simulink model "TP9_commande_ceintures_airbags"  (R2022b)
settings: Solver=VariableStepAuto  StartTime=0.0  StopTime=inf  RelTol=1e-3
libraries: dspsnks4 x2
settings Model: Creator=HP  LastModifiedBy=HP

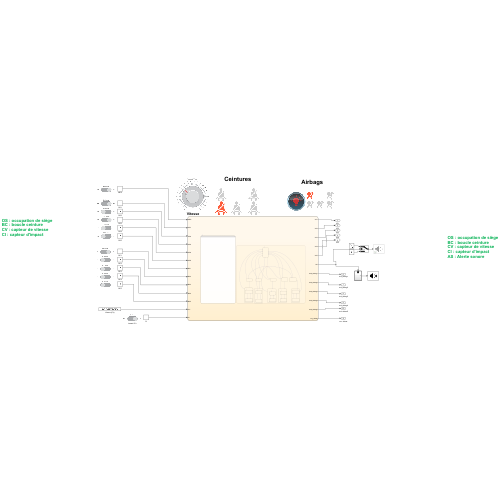
[thumbnail: Simulink's stored preview of the top-level diagram]
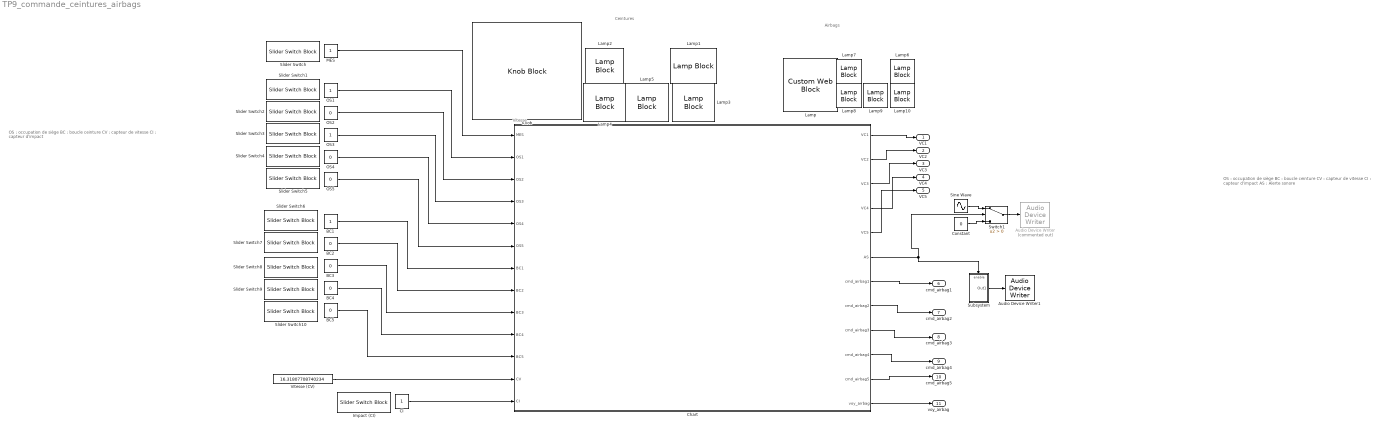
== system TP9_commande_ceintures_airbags ==
  note: Ceintures
  note: OS : occupation de siège
      | BC : boucle ceinture
      | CV : capteur de vitesse
      | CI : capteur d'impact
  note: OS : occupation de siège
      | BC : boucle ceinture
      | CV : capteur de vitesse
      | CI : capteur d'impact
      | AS : Alerte sonore
  note: Airbags
  note: Vitesse
  Audio Device Writer : dspsnks4/Audio Device Writer  Commented=on  Driver=DirectSound  Device=Default  InheritSampleRate=on  SampleRate=44100  BitDepth=16-bit integer  BufferSize=4096  NumBuffers=10  DefaultOutputChannelMapping=on  OutputChannelMapping=1:2  OutputNumUnderrunSamples=off  DriverIdx=1  DeviceWarnFlag=''
  Audio Device Writer1 : dspsnks4/Audio Device Writer  Driver=DirectSound  Device=Default  InheritSampleRate=on  SampleRate=44100  BitDepth=16-bit integer  BufferSize=4096  NumBuffers=10  DefaultOutputChannelMapping=on  OutputChannelMapping=1:2  OutputNumUnderrunSamples=off  DriverIdx=1  DeviceWarnFlag=''
  BC1 : Constant
  BC{2..5} (4 alike) : Constant  Value=0
  CI : Constant
  Chart : Stateflow chart  TreatAsAtomicUnit=on
      settings: PortSchema="{\"entries\":[{\"content\":{\"sides\":[{\"content\":{\"connectorIds\":[\"In1\",\"In2\",\"In3\",\"In4\",\"In5\",\"In6\",\"In7\",\"In8\",\"In9\",\"In10\",\"In12\",\"In11\",\"In13\"]},\"type\":\"ConnectorPlacement.EquallySpacedRectSide\",\"uuid\":\"46ff6330-a002-4d17-9cd2-f1bd6e651efc\"},{\"content\":{\"connectorIds\":[\"Out1\",\"Out2\",\"Out3\",\"Out4\",\"Out5\",\"Out6\",\"Out7\",\"Out8\",\"Out9\",\"Out10\",\"Out11\",\"Out12\"],\"side\":\"RIGHT\"},\"type\":\"ConnectorPlacement.EquallySpacedRectSide\",\"uuid\":\"880f7646-c9e2-4dea-b189-cc9f9386497e\"},{\"content\":{\"connectorIds\":[],\"side\":\"TOP\"},\"type\":\"ConnectorPlacement.EquallySpacedRectSide\",\"uuid\":\"9bbd1801-2f42-4ba2-a8a0-b1f6ca3d8990\"}]},\"type\":\"ConnectorPlacement.EquallySpacedConnector\",\"uuid\":\"8416df3d-9e50-44e6-a163-5e155c7c1857\"}],\"packageUris\":[\"http://schema.mathworks.com/mf0/Connector/R2020b\"],\"version\":\"1.0\"}"
  Constant : Constant  Value=0
  Impact (CI) : SliderSwitchBlock
      settings: Values={{'Off', 'On'}, [0 1]}
  Knob : KnobBlock  ScaleMax=50
  Lamp : CustomWebBlock  LabelPosition=Hide  ShowInitialText=on  Configuration="{\"components\":[{\"name\":\"BackgroundImageComponent\",\"settings\":{\"image\":{\"size\":[150,150],\"src\":\"data:image\\/svg+xml;base64,PHN2ZyB4bWxucz0iaHR0cDovL3d3dy53My5vcmcvMjAwMC9zdmciIHhtbG5zOnhsaW5rPSJodHRwOi8vd3d3LnczLm9yZy8xOTk5L3hsaW5rIiB2aWV3Qm94PSIwIDAgNTAwIDUwMCI+PGRlZnM+PHN0eWxlPi5he2ZpbGw6dXJsKCNhKTt9LmJ7ZmlsbDp1cmwoI2IpO30uY3tmaWxsOnVybCgjYyk7fTwvc3R5bGU+PHJhZGlhbEdyYWRpZW50IGlkPSJhIiBjeD0iMjgzLjg0IiBjeT0iLTQ2Ni4zNyIgcj0iMzc1Ljc1IiBncmFkaWVudFRyYW5zZm9ybT0ibWF0cml4KDEuMzksIDAsIDAsIC0xLjM5LCAtMTUzLjU2LCAtNjQ0LjA4KSIg ...(+2088 chars)\",\"srcOrientation\":\"Right\"},\"position\":[0,0,1,1],\"scaleMode\":\"0\"}},{\"name\":\"LampStateComponent\",\"settings\":{\"position\":[0,0,1,1],\"states\":[{\"icon\":{\"customSrc\":\"data:image\\/svg+xml;base64,PHN2ZyBpZD0iTGF5ZXJfMSIgZGF0YS1uYW1lPSJMYXllciAxIiB4bWxucz0iaHR0cDovL3d3dy53My5vcmcvMjAwMC9zdmciIHZpZXdCb3g9IjAgMCA0MTEgNDU4Ij48ZGVmcz48c3R5bGU+LmNscy0xe2ZpbGw6I2ZkZjhjMTt9LmNscy0ye2ZpbGw6I2ZlZTEwMDt9LmNscy0ze2ZpbGw6IzIzMWYyMDt9LmNscy00e2ZpbGw6I2EwOWY5Zjt9LmNscy00LC5jbHMtNSwuY2xzLTZ7c3Ryb2tlOiMyMzFmMjA7c3Ryb2tlLW1pdGVybGltaXQ6MTA7fS5jbHMtNXtmaWxsOiNmZmY7fS5jbHMtNntmaWxsOm5vbmU7fTwvc3R5bGU+PC9kZWZz ...(+5168 chars)\",\"id\":-1,\"srcOrientation\":\"Right\",\"type\":\"custom\"},\"iconScale\":0.8,\"metadata\":{},\"overlayType\":\"intersect\",\"shape\":{\"color\":[0.725,0,0],\"opacity\":1,\"position\":[0.1,0.1,0.8,0.8],\"type\":\"ellipse\"},\"value\":[]},{\"icon\":{\"customSrc\":\"data:image\\/svg+xml;base64,PHN2ZyBpZD0iTGF5ZXJfMSIgZGF0YS1uYW1lPSJMYXllciAxIiB4bWxucz0iaHR0cDovL3d3dy53My5vcmcvMjAwMC9zdmciIHZpZXdCb3g9IjAgMCA0MTEgNDU4Ij48ZGVmcz48c3R5bGU+LmNscy0xe2ZpbGw6I2ZkZjhjMTt9LmNscy0ye2ZpbGw6I2ZlZTEwMDt9LmNscy0ze2ZpbGw6IzIzMWYyMDt9LmNscy00e2ZpbGw6I2EwOWY5Zjt9LmNscy00LC5jbHMtNSwuY2xzLTZ7c3Ryb2tlOiMyMzFmMjA7c3Ryb2tlLW1pdGVybGltaXQ6MTA7fS5jbHMtNXtmaWxsOiNmZmY7fS5jbHMtNntmaWxsOm5vbmU7fTwvc3R5bGU+PC9kZWZz ...(+5168 chars)\",\"id\":-1,\"srcOrientation\":\"Right\",\"type\":\"custom\"},\"iconScale\":0.8,\"metadata\":{\"useDefaults\":{\"customIcon\":true,\"icon\":true,\"overlayType\":true,\"shape\":true,\"sizeAndPosition\":true}},\"overlayType\":\"intersect\",\"shape\":{\"color\":[0,0,0],\"opacity\":1,\"position\":[0.1,0.1,0.8,0.8],\"type\":\"ellipse\"},\"value\":\"0\"}],\"valueType\":\"discrete\"}},{\"name\":\"ForegroundImageComponent\",\"settings\":{\"image\":{\"size\":[150,150],\"src\":\"data:image\\/svg+xml;base64,PHN2ZyB4bWxucz0iaHR0cDovL3d3dy53My5vcmcvMjAwMC9zdmciIHhtbG5zOnhsaW5rPSJodHRwOi8vd3d3LnczLm9yZy8xOTk5L3hsaW5rIiB2aWV3Qm94PSIwIDAgNTAwIDUwMCI+PGRlZnM+PHN0eWxlPi5he2ZpbGw6dXJsKCNhKTt9PC9zdHlsZT48bGluZWFyR3JhZGllbnQgaWQ9ImEiIHgxPSIxNzMuMDUiIHkxPSItNjI3Ljc4IiB4Mj0iMTczLjA1IiB5Mj0iLTUyMi40MyIgZ3JhZGllbnRUcmFuc2Zvcm09Im1hdHJpeCgxLjI5LCAwLCAwLCAtMS4zMywgMjcuMTMsIC02MjguMzEpIiBncmFkaWVudFVuaXRzPSJ1c2VyU3BhY2VPblVzZSI+PHN0b3Agb2Zmc2V0PSIwIiBzdG9wLWNvbG9yPSIjZmZmIiBzdG9wLW9wYWNpdHk9IjAuMjUiLz48c3RvcCBvZmZzZXQ9IjEiIHN0b3AtY29sb3I9IiNmZmYiIHN0b3Atb3BhY2l0eT0iMCIvPjwvbGluZWFyR3JhZGllbnQ+PC9kZWZzPjxwYXRoIGNsYXNzPSJhIiBkPSJNNDI5LjMsMTkwLjY2QzQwMi40NSwxMTQuNTEsMzMyLjY3LDYwLjE3LDI1MC44NSw2MC4xN2MtODMuNDMsMC0xNTQuMjgsNTYuNDItMTc5Ljk1LDEzNSwxNS4zNCwzOSw4OC4xMSw3LDE3Ny4wNyw3QzM0MCwyMDIuMDgsNDE3LjI2LDIzNi40Niw0MjkuMywxOTAuNjZaIi8+PC9zdmc+\",\"srcOrientation\":\"Right\"},\"isForeground\":1,\"position\":[0,0,1,1],\"scaleMode\":\"0\"}}],\"settings\":{\"BindingType\":\"signal\",\"aspectRatio\":1.032258064516129,\"backgroundColor\":[0,0,0],\"backgroundOffset\":0.14,\"backgroundOpacity\":1,\"blockOrientation\":\"Right\",\"fixedAspectRatio\":\"on\",\"showBackgroundColor\":false,\"value\":0,\"version\":\"22a\"},\"type\":\"Lamp\"}"
  Lamp{1..5} (5 alike) : LampBlock  LabelPosition=Hide  Icon=Custom  CustomIcon=data:image/svg+xml;base64,PD94bWwgdmVyc2lvbj0iMS4wIiBzdGFuZGFsb25lPSJubyI/Pgo8IURPQ1RZUEUgc3ZnIFBVQkxJQyAiLS8vVzNDLy9EVEQgU1ZHIDIwMDEwOTA0Ly9FTiIKICJodHRwOi8vd3d3LnczLm9yZy9UUi8yMDAxL1JFQy1TVkctMjAwMTA5MDQvRFREL3N2ZzEwLmR0ZCI+CjxzdmcgdmVyc2lvbj0iMS4wIiB4bWxucz0iaHR0cDovL3d3dy53My5vcmcvMjAwMC9zdmciCiB3aWR0aD0iNDU5LjAwMDAwMHB0IiBoZWlnaHQ9IjU0My4wMDAwMDBwdCIgdmlld0JveD0iMCAwIDQ1OS4wMDAwMDAgNTQzLjAwMDAwMCIKIHByZXNlcnZlQXNwZWN0 ...(+2800 chars)
  Lamp{6..10} (5 alike) : LampBlock  LabelPosition=Hide  Icon=Custom  CustomIcon=data:image/svg+xml;base64,PD94bWwgdmVyc2lvbj0iMS4wIiBzdGFuZGFsb25lPSJubyI/Pgo8IURPQ1RZUEUgc3ZnIFBVQkxJQyAiLS8vVzNDLy9EVEQgU1ZHIDIwMDEwOTA0Ly9FTiIKICJodHRwOi8vd3d3LnczLm9yZy9UUi8yMDAxL1JFQy1TVkctMjAwMTA5MDQvRFREL3N2ZzEwLmR0ZCI+CjxzdmcgdmVyc2lvbj0iMS4wIiB4bWxucz0iaHR0cDovL3d3dy53My5vcmcvMjAwMC9zdmciCiB3aWR0aD0iNTIxLjAwMDAwMHB0IiBoZWlnaHQ9IjQ3OS4wMDAwMDBwdCIgdmlld0JveD0iMCAwIDUyMS4wMDAwMDAgNDc5LjAwMDAwMCIKIHByZXNlcnZlQXNwZWN0 ...(+2508 chars)
  MES : Constant
  OS1 : Constant
  OS2 : Constant  Value=0
  OS3 : Constant
  OS4 : Constant  Value=0
  OS5 : Constant  Value=0
  Sine Wave : Sin  Frequency=2*pi*1000  SampleTime=1/48000
  Slider Switch{,1..10} (11 alike) : SliderSwitchBlock
      settings: Values={{'Off', 'On'}, [0 1]}
  Subsystem : Subsystem
  Switch1 : Switch  Criteria=u2 > Threshold  SaturateOnIntegerOverflow=off  InputSameDT=off
  Vitesse (CV) : Constant  Value=16.31807708740234
  VC1 : Outport
  VC2 : Outport  Port=2
  VC3 : Outport  Port=3
  VC4 : Outport  Port=4
  VC5 : Outport  Port=5
  cmd_airbag1 : Outport  Port=6
  cmd_airbag2 : Outport  Port=7
  cmd_airbag3 : Outport  Port=8
  cmd_airbag4 : Outport  Port=9
  cmd_airbag5 : Outport  Port=10
  voy_airbag : Outport  Port=11
  wires:
  MES/1 -> Chart/1(MES)
  OS1/1 -> Chart/2(OS1)
  OS2/1 -> Chart/3(OS2)
  OS3/1 -> Chart/4(OS3)
  OS4/1 -> Chart/5(OS4)
  OS5/1 -> Chart/6(OS5)
  BC1/1 -> Chart/7(BC1)
  BC2/1 -> Chart/8(BC2)
  BC3/1 -> Chart/9(BC3)
  BC4/1 -> Chart/10(BC4)
  BC5/1 -> Chart/12(BC5)
  Vitesse (CV)/1 -> Chart/11(CV)
  Chart/1(VC1) -> VC1/1
  Chart/2(VC2) -> VC2/1
  Chart/3(VC3) -> VC3/1
  Chart/4(VC4) -> VC4/1
  Chart/5(VC5) -> VC5/1
  Chart/6(AS) -> Switch1/2, Subsystem/Enable
  Constant/1 -> Switch1/3
  Switch1/1 -> Audio Device Writer/1
  Sine Wave/1 -> Switch1/1
  Subsystem/1(Out1) -> Audio Device Writer1/1
  CI/1 -> Chart/13(CI)
  Chart/7(cmd_airbag1) -> cmd_airbag1/1
  Chart/8(cmd_airbag2) -> cmd_airbag2/1
  Chart/9(cmd_airbag3) -> cmd_airbag3/1
  Chart/11(cmd_airbag5) -> cmd_airbag5/1
  Chart/10(cmd_airbag4) -> cmd_airbag4/1
  Chart/12(voy_airbag) -> voy_airbag/1

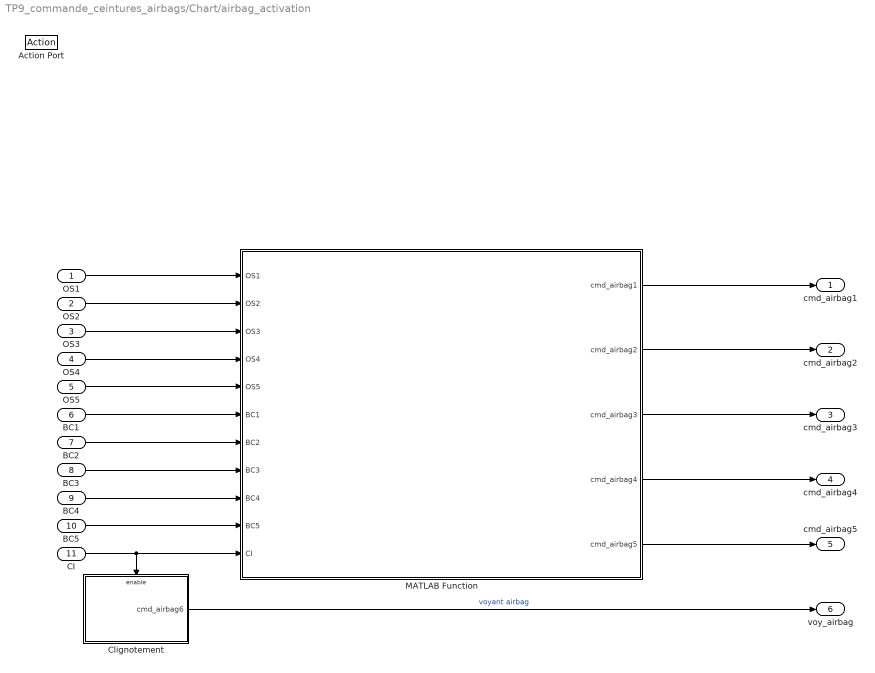
== system TP9_commande_ceintures_airbags/Chart/airbag_activation ==
  OS1 : Inport
  OS2 : Inport  Port=2
  OS3 : Inport  Port=3
  OS4 : Inport  Port=4
  OS5 : Inport  Port=5
  BC1 : Inport  Port=6
  BC2 : Inport  Port=7
  BC3 : Inport  Port=8
  BC4 : Inport  Port=9
  BC5 : Inport  Port=10
  CI : Inport  Port=11
  Action Port : ActionPort
      settings: CopyFcn=Stateflow.SLINSF.SimulinkMan.removeBlockPreDeleteFcn  PreDeleteFcn=Stateflow.SLINSF.SimulinkMan.unsafePredeleteFcn
  Clignotement : Subsystem
  MATLAB Function : MATLAB Function  TreatAsAtomicUnit=on
  cmd_airbag1 : Outport
  cmd_airbag2 : Outport  Port=2
  cmd_airbag3 : Outport  Port=3
  cmd_airbag4 : Outport  Port=4
  cmd_airbag5 : Outport  Port=5
  voy_airbag : Outport  Port=6
  wires:
  MATLAB Function/1(cmd_airbag1) -> cmd_airbag1/1
  OS1/1 -> MATLAB Function/1(OS1)
  OS2/1 -> MATLAB Function/2(OS2)
  OS3/1 -> MATLAB Function/3(OS3)
  OS4/1 -> MATLAB Function/4(OS4)
  OS5/1 -> MATLAB Function/5(OS5)
  BC1/1 -> MATLAB Function/6(BC1)
  BC2/1 -> MATLAB Function/7(BC2)
  BC3/1 -> MATLAB Function/8(BC3)
  BC4/1 -> MATLAB Function/9(BC4)
  BC5/1 -> MATLAB Function/10(BC5)
  CI/1 -> Clignotement/Enable, MATLAB Function/11(CI)
  Clignotement/1(cmd_airbag6) -> voy_airbag/1  "voyant airbag"
  MATLAB Function/2(cmd_airbag2) -> cmd_airbag2/1
  MATLAB Function/3(cmd_airbag3) -> cmd_airbag3/1
  MATLAB Function/4(cmd_airbag4) -> cmd_airbag4/1
  MATLAB Function/5(cmd_airbag5) -> cmd_airbag5/1

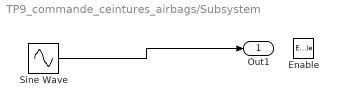
== system TP9_commande_ceintures_airbags/Subsystem ==
  Enable : EnablePort
  Sine Wave : Sin  Frequency=2*pi*1000  SampleTime=1/48000
  Out1 : Outport
  wires:
  Sine Wave/1 -> Out1/1

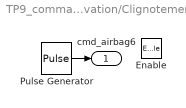
== system TP9_commande_ceintures_airbags/Chart/airbag_activation/Clignotement ==
  Enable : EnablePort
  Pulse Generator : DiscretePulseGenerator  Period=10  PulseWidth=5  SampleTime=0.1
  cmd_airbag6 : Outport
  wires:
  Pulse Generator/1 -> cmd_airbag6/1

== matlab function TP9_commande_ceintures_airbags/Chart/airbag_activation/MATLAB Function ==
  data: cmd_airbag1 output; OS1 input; OS2 input; OS3 input; OS4 input; OS5 input; BC1 input; BC2 input; BC3 input; BC4 input; BC5 input; CI input; cmd_airbag2 output; cmd_airbag3 output; cmd_airbag4 output; cmd_airbag5 output
function [cmd_airbag1, cmd_airbag2, cmd_airbag3, cmd_airbag4, cmd_airbag5] = airbag(OS1, OS2, OS3, OS4, OS5, BC1, BC2, BC3, BC4, BC5, CI)

if (CI == 1 && OS1 == 1 && BC1 == 1)
    cmd_airbag1 = 1;
else
    cmd_airbag1 = 0;
end    


if (CI == 1 && OS2 == 1 && BC2 == 1)
    cmd_airbag2 = 1;
else
    cmd_airbag2 =0;
end


if (CI == 1 && OS3 == 1 && BC3 == 1)
   cmd_airbag3 = 1;
else
    cmd_airbag3 =0;
end


if (CI == 1 && OS4 == 1 && BC4 == 1)
    cmd_airbag4 = 1;
else
    cmd_airbag4 =0;
end


if (CI == 1 && OS5 == 1 && BC5 == 1)
    cmd_airbag5 = 1;
else
    cmd_airbag5 =0;
end

== stateflow chart TP9_commande_ceintures_airbags/Chart ==
  settings: updateMethod=DISCRETE  sampleTime=0.1
  state airbag_activation [parallel]
    settings: executionOrder=2
  state gestion_ceintures [parallel]
    settings: executionOrder=1
    state REPOS
      VC1 = 0;
      VC2 = 0;
      VC3 = 0;
      VC4 = 0;
      VC5 = 0;
      AS = 0;
    state SIEGE4_OCCUPE
      entry:
      VC4 = 1;
      AS = 0;
    state SIEGE5_OCCUPE
      entry:
      VC5 = 1;
      AS = 0;
    state SIEGE3_OCCUPE
      entry:
      VC3 = 1;
      AS = 0;
    state SIEGE2_OCCUPE
      VC2 = 1;
      AS = 0;
    state SIEGE1_OCCUPE
      VC1 = 1;
      AS = 0;
    state bip1
      state SIEGE1_OCCUPE1
        entry:
        VC1 = 1;
        AS = 1;
      state SIEGE1_OCCUPE2
        entry:
        VC1 = 1;
        AS = 0;
      (default) -> SIEGE1_OCCUPE1
      SIEGE1_OCCUPE1 -> SIEGE1_OCCUPE2 : [after(1, sec)]
      SIEGE1_OCCUPE2 -> SIEGE1_OCCUPE1 : [after(1, sec)]
    state bip2
      state SIEGE2_OCCUPE1
        VC2 = 1;
        AS = 1;
      state SIEGE2_OCCUPE2
        VC2 = 1;
        AS = 0;
      (default) -> SIEGE2_OCCUPE1
      SIEGE2_OCCUPE1 -> SIEGE2_OCCUPE2 : [after(1, sec)]
      SIEGE2_OCCUPE2 -> SIEGE2_OCCUPE1 : [after(1, sec)]
    state bip3
      state SIEGE3_OCCUPE1
        VC3 = 1;
        AS = 1;
      state SIEGE3_OCCUPE2
        VC3 = 1;
        AS = 0;
      (default) -> SIEGE3_OCCUPE1
      SIEGE3_OCCUPE1 -> SIEGE3_OCCUPE2 : [after(1, sec)]
      SIEGE3_OCCUPE2 -> SIEGE3_OCCUPE1 : [after(1, sec)]
    state bip4
      state SIEGE4_OCCUPE1
        VC4 = 1;
        AS = 1;
      state SIEGE4_OCCUPE2
        VC4 = 1;
        AS = 0;
      (default) -> SIEGE4_OCCUPE1
      SIEGE4_OCCUPE1 -> SIEGE4_OCCUPE2 : [after(1, sec)]
      SIEGE4_OCCUPE2 -> SIEGE4_OCCUPE1 : [after(1, sec)]
    state bip5
      state SIEGE5_OCCUPE1
        VC5 = 1;
        AS = 1;
      state SIEGE5_OCCUPE2
        VC5 = 1;
        AS = 0;
      SIEGE5_OCCUPE1 -> SIEGE5_OCCUPE2 [order 2] : [after(1, sec)]
      SIEGE5_OCCUPE2 -> SIEGE5_OCCUPE1 : [after(1, sec)]
    (default) -> REPOS
    bip1 -> REPOS : [MES == 0 || BC1 == 1 || OS1 == 0]
    SIEGE1_OCCUPE -> REPOS [order 2] : [MES == 0 || BC1 == 1 || OS1 == 0]
    SIEGE5_OCCUPE1 -> REPOS [order 1] : [MES == 0 || BC5 == 1 || OS5 == 0]
    SIEGE2_OCCUPE -> REPOS [order 2] : [MES == 0 || BC2 == 1 || OS2 == 0]
    SIEGE5_OCCUPE -> REPOS [order 2] : [MES == 0 || BC5 == 1 || OS5 == 0]
    SIEGE4_OCCUPE -> REPOS [order 2] : [MES == 0 || BC4 == 1 || OS4 == 0]
    bip2 -> REPOS : [MES == 0 || BC2 == 1 || OS2 == 0]
    bip4 -> REPOS : [MES == 0 || BC4 == 1 || OS4 == 0]
    SIEGE3_OCCUPE -> REPOS [order 2] : [MES == 0 || BC3 == 1 || OS3 == 0]
    bip3 -> REPOS : [MES == 0 || BC3 == 1 || OS3 == 0]
    REPOS -> (junction 25) : [MES == 1]
    (junction 25) -> SIEGE1_OCCUPE [order 1] : [OS1 == 1 && BC1 == 0]
    (junction 25) -> SIEGE5_OCCUPE [order 5] : [OS5 == 1 && BC5 == 0]
    (junction 25) -> SIEGE4_OCCUPE [order 4] : [OS4 == 1 && BC4 == 0]
    (junction 25) -> SIEGE2_OCCUPE [order 2] : [OS2 == 1 && BC2 == 0]
    (junction 25) -> SIEGE3_OCCUPE [order 3] : [OS3 == 1 && BC3 == 0]
    SIEGE5_OCCUPE -> SIEGE5_OCCUPE1 [order 1] : [(CV >= 15 && (OS5 == 1 && BC5 == 0)) || (CV< 15 && OS5 == 1 && BC5 == 0 && after(60, sec))]
    SIEGE1_OCCUPE -> bip1 [order 1] : [(CV >= 15 && (OS1== 1 && BC1 == 0)) || (CV< 15 && OS1 == 1 && BC1 == 0 && after(60, sec))]
    SIEGE2_OCCUPE -> bip2 [order 1] : [(CV >= 15 && (OS2 == 1 && BC2 == 0)) || (CV< 15 && OS2 == 1 && BC2 == 0 && after(60, sec))]
    SIEGE3_OCCUPE -> bip3 [order 1] : [(CV >= 15 && (OS3 == 1 && BC3 == 0)) || (CV< 15 && OS3 == 1 && BC3 == 0 && after(60, sec))]
    SIEGE4_OCCUPE -> bip4 [order 1] : [(CV >= 15 && (OS4 == 1 && BC4 == 0)) || (CV< 15 && OS4 == 1 && BC4 == 0 && after(60, sec))]
  (default) -> airbag_activation
  data: sf_internal_action_state_placeholder_data local double size=1 =0; MES input; OS1 input; OS2 input; OS3 input; OS4 input; OS5 input; BC1 input; BC2 input; BC3 input; BC4 input; CV input; BC5 input; VC1 output; VC2 output; VC3 output; VC4 output; VC5 output; AS output; CI input; cmd_airbag1 output double size=1; cmd_airbag2 output; cmd_airbag3 output; cmd_airbag4 output; cmd_airbag5 output; data local; voy_airbag output
